simulink model "yuan_untitled_final_waveforms_SOM_PLL_fixed"  (R2023b)
settings: Solver=FixedStepDiscrete  StartTime=0.0  StopTime=0.5  FixedStep=1e-6  RelTol=1e-3
libraries: slpidlib x3, spsDCVoltageSourceLib x1, spsGroundLib x1, spsPermanentMagnetSynchronousMachineLib x1, spsThreePhaseVIMeasurementLib x1, spsUniversalBridgeLib x1, sps_lib x1
settings Model: Creator=zxw  LastModifiedBy=zxw

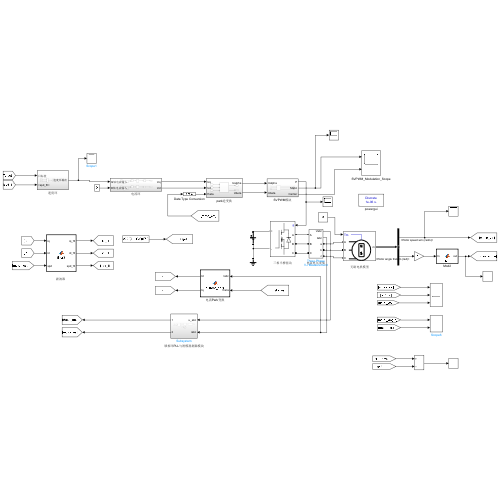
[thumbnail: Simulink's stored preview of the top-level diagram]
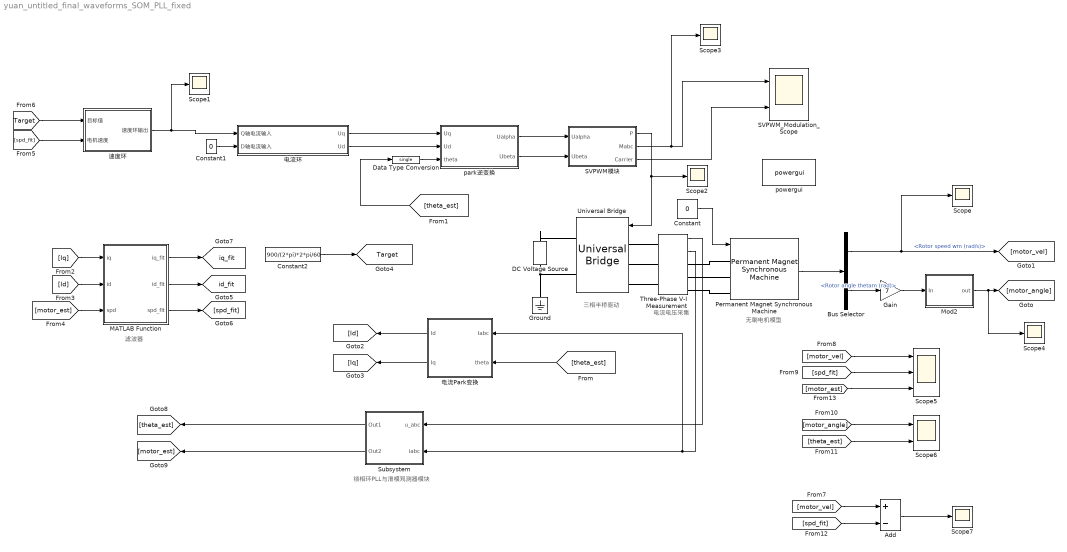
== system yuan_untitled_final_waveforms_SOM_PLL_fixed ==
  note: 锁相环PLL与滑模观测器模块
  note: 滤波器
  note: 无刷电机模型
  note: 电流电压采集
  note: 三相半桥驱动
  Add : Sum  Inputs=+-
  Bus Selector : BusSelector  OutputSignals=Rotor speed wm (rad/s),Rotor angle thetam (rad)
  Constant : Constant  Value=0
  Constant1 : Constant  Value=0
  Constant2 : Constant  Value=900/(2*pi)*2*pi/60
  DC Voltage Source : spsDCVoltageSourceLib/DC Voltage Source  Amplitude=24  Measurements=None
  Data Type Conversion : DataTypeConversion  OutDataTypeStr=single  RndMeth=Nearest  SaturateOnIntegerOverflow=off
  Gain : Gain  Gain=7
  Ground : spsGroundLib/Ground  LConnTagsString=a
  MATLAB Function : MATLAB Function  TreatAsAtomicUnit=on
  Mod2 : MATLAB Function  TreatAsAtomicUnit=on
  Permanent Magnet Synchronous Machine : spsPermanentMagnetSynchronousMachineLib/Permanent Magnet Synchronous Machine  NbPhases=3  FluxDistribution=Sinusoidal  RotorType=Round  MechanicalLoad=Torque Tm  PresetModel=No  ShowDetailedParameters=on  MeasurementBus=off  Resistance=0.0485  Inductance=8.5e-3  dqInductances=[8.5e-3,8.5e-3]  La=0.000395  MachineConstant=Flux linkage established by magnets (V.s)  Flux=0.1194  VoltageCst=151.5974  TorqueCst=1.2537  Flat=120  Mechanical=[0.0027 0.0004924 7 0]  PolePairs=4  InitialConditions=[0,0, 0,0]  InitialConditions5ph=[0 0 0 0 0 0]  RefAngle=90 degrees behind phase A axis (modified Park)  IterativeDiscreteModel=Trapezoidal non iterative  TsBlock=-1  TsPowergui=0
  SVPWM_Modulation_Scope : Scope  NumInputPorts=2
  SVPWM模块 : Subsystem
  Scope{,1..4,7} (6 alike) : Scope
  Scope5 : Scope  NumInputPorts=3
  Scope6 : Scope  NumInputPorts=2
  Subsystem : Subsystem
  Three-Phase V-I Measurement : spsThreePhaseVIMeasurementLib/Three-Phase V-I Measurement  VoltageMeasurement=phase-to-ground  SetLabelV=off  LabelV=Vabc  Vpu=off  VpuLL=off  CurrentMeasurement=yes  SetLabelI=off  LabelI=Iabc  Ipu=off  Pbase=100e6  Vbase=500e3  OutputType=Complex  PhasorSimulation=off  PSBequivalent=0
  Universal Bridge : spsUniversalBridgeLib/Universal Bridge  Arms=3  SnubberResistance=1e5  SnubberCapacitance=inf  Device=MOSFET / Diodes  Ron=1e-3  Lon=0  ForwardVoltages="[  0  0  ]"  ForwardVoltage=0  GTOparameters=[ 10e-6 , 20e-6 ]  IGBTparameters=[ 1e-6 , 2e-6 ]  Measurements=None  Measurements_2=None  converterType=Rectifier
  park逆变换 : Subsystem
  powergui : sps_lib/powergui  Priority=1  SimulationMode=Discrete  SampleTime=1e-6  frequency=60  Iterations=50  frequencyindice=0  Pbase=100e6  ErrMax=1e-4  UnitsV=kV  UnitsW=MW  buscounter=0  FunctionMessages=off  echomessages=off  EnableUseOfTLC=off  CurrentSourceSwitches=off  DisableSnubberDevices=off  DisableRonSwitches=off  DisableVfSwitches=off  DisplayEquations=off  AutomaticDiscreteSolvers=off  SolverType=Tustin/Backward Euler (TBE)  Interpol=off  ExternalGateDelay=off  methode=off  Ts=100  x0status=blocks  SPID=on  SwTol=0  HookPort=off  NonlinearTolerance=1e-4  nMaxIteration=100  ContinueOnMaxIteration=off  RestoreLinks=warning  ResistiveCurrentMeasurement=off  Frange=[0:2:500]  Ylog=off  Xlog=on  ShowGrid=off  save=off  variable=ZData  structure=0  ZoomFFT=off  StartTime=0.0  cycles=1  DisplayStyle=1  fundamental=60  FreqAxis=off  MaxFrequency=1000  frequencyindicesteady=1  RmsSteady=1  display=off
  电流Park变换 : MATLAB Function  TreatAsAtomicUnit=on
  电流环 : Subsystem
  速度环 : Subsystem
  tag scope: Target=global, id_fit=global, iq_fit=global
  wires:
  Permanent Magnet Synchronous Machine/1 -> Bus Selector/1
  Bus Selector/2 -> Gain/1  "<Rotor angle thetam (rad)>"
  Gain/1 -> Mod2/1(In)
  Mod2/1(out) -> Scope4/1, [motor_angle]
  Bus Selector/1 -> Scope/1, [motor_vel]  "<Rotor speed wm (rad/s)>"
  Constant/1 -> Permanent Magnet Synchronous Machine/1
  park逆变换/2(Ubeta) -> SVPWM模块/2(Ubeta)
  park逆变换/1(Ualpha) -> SVPWM模块/1(Ualpha)
  [theta_est] -> 电流Park变换/2(theta)
  Data Type Conversion/1 -> park逆变换/3(theta)
  [theta_est] -> Data Type Conversion/1
  电流Park变换/1(Id) -> [Id]
  电流Park变换/2(Iq) -> [Iq]
  [Iq] -> MATLAB Function/1(iq)
  [Id] -> MATLAB Function/2(id)
  [motor_est] -> MATLAB Function/3(spd)
  MATLAB Function/1(iq_flt) -> [iq_fit]
  MATLAB Function/2(id_flt) -> [id_fit]
  MATLAB Function/3(spd_flt) -> [spd_fit]
  电流环/2(Ud) -> park逆变换/2(Ud)
  电流环/1(Uq) -> park逆变换/1(Uq)
  Constant1/1 -> 电流环/2(D轴电流输入)
  Constant2/1 -> [Target]
  [Target] -> 速度环/1(目标值)
  [spd_fit] -> 速度环/2(电机速度)
  速度环/1(速度环输出) -> Scope1/1, 电流环/1(Q轴电流输入)
  SVPWM模块/2(Mabc) -> Scope3/1, SVPWM_Modulation_Scope/1
  SVPWM模块/3(Carrier) -> SVPWM_Modulation_Scope/2
  SVPWM模块/1(P) -> Scope2/1, Universal Bridge/1
  Three-Phase V-I Measurement/2 -> 电流Park变换/1(Iabc), Subsystem/2(iabc)
  [motor_vel] -> Scope5/1
  [spd_fit] -> Scope5/2
  [theta_est] -> Scope6/2
  [motor_angle] -> Scope6/1
  Three-Phase V-I Measurement/1 -> Subsystem/1(u_abc)
  Subsystem/1(Out1) -> [theta_est]
  Subsystem/2(Out2) -> [motor_est]
  [spd_fit] -> Add/2
  [motor_vel] -> Add/1
  Add/1 -> Scope7/1
  [motor_est] -> Scope5/3
  connections:
  Three-Phase V-I Measurement/RConn1 -- Permanent Magnet Synchronous Machine/LConn1
  Three-Phase V-I Measurement/RConn2 -- Permanent Magnet Synchronous Machine/LConn2
  Three-Phase V-I Measurement/RConn3 -- Permanent Magnet Synchronous Machine/LConn3
  Universal Bridge/LConn1 -- Three-Phase V-I Measurement/LConn1
  Universal Bridge/LConn2 -- Three-Phase V-I Measurement/LConn2
  Universal Bridge/LConn3 -- Three-Phase V-I Measurement/LConn3
  DC Voltage Source/RConn1 -- Universal Bridge/RConn1
  DC Voltage Source/LConn1 -- Universal Bridge/RConn2 -- Ground/LConn1

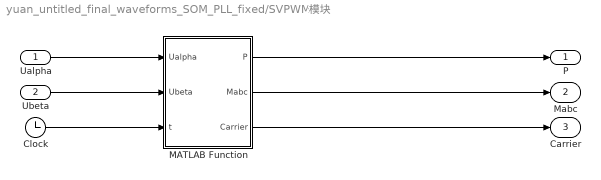
== system yuan_untitled_final_waveforms_SOM_PLL_fixed/SVPWM模块 ==
  Ualpha : Inport
  Ubeta : Inport  Port=2
  Clock : Clock
  MATLAB Function : MATLAB Function  TreatAsAtomicUnit=on
  P : Outport
  Mabc : Outport  Port=2
  Carrier : Outport  Port=3
  wires:
  Ualpha/1 -> MATLAB Function/1(Ualpha)
  MATLAB Function/1(P) -> P/1
  Ubeta/1 -> MATLAB Function/2(Ubeta)
  Clock/1 -> MATLAB Function/3(t)
  MATLAB Function/2(Mabc) -> Mabc/1
  MATLAB Function/3(Carrier) -> Carrier/1

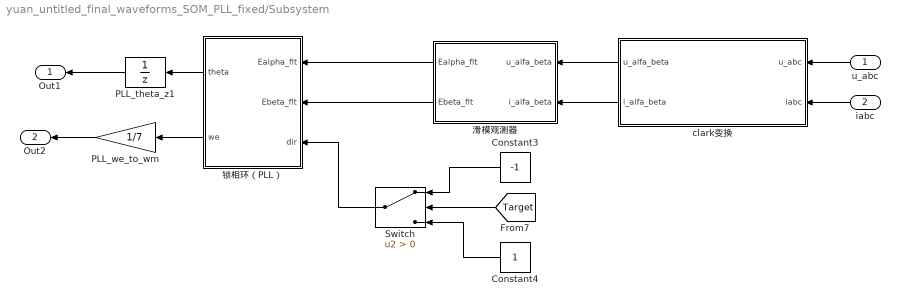
== system yuan_untitled_final_waveforms_SOM_PLL_fixed/Subsystem ==
  u_abc : Inport
  iabc : Inport  Port=2
  Constant3 : Constant  Value=-1
  Constant4 : Constant
  PLL_theta_z1 : UnitDelay  SampleTime=1e-6  HasFrameUpgradeWarning=on
  PLL_we_to_wm : Gain  Gain=1/7
  Switch : Switch  Criteria=u2 > Threshold  SaturateOnIntegerOverflow=off  InputSameDT=off
  clark变换 : MATLAB Function  TreatAsAtomicUnit=on
  滑模观测器 : MATLAB Function  TreatAsAtomicUnit=on
  锁相环（PLL） : MATLAB Function  TreatAsAtomicUnit=on
  Out1 : Outport
  Out2 : Outport  Port=2
  wires:
  PLL_we_to_wm/1 -> Out2/1
  clark变换/2(i_alfa_beta) -> 滑模观测器/2(i_alfa_beta)
  clark变换/1(u_alfa_beta) -> 滑模观测器/1(u_alfa_beta)
  滑模观测器/2(Ebeta_flt) -> 锁相环（PLL）/2(Ebeta_flt)
  Constant3/1 -> Switch/1
  滑模观测器/1(Ealpha_flt) -> 锁相环（PLL）/1(Ealpha_flt)
  Constant4/1 -> Switch/3
  Switch/1 -> 锁相环（PLL）/3(dir)
  [Target] -> Switch/2
  锁相环（PLL）/1(theta) -> PLL_theta_z1/1
  锁相环（PLL）/2(we) -> PLL_we_to_wm/1
  PLL_theta_z1/1 -> Out1/1
  iabc/1 -> clark变换/2(iabc)
  u_abc/1 -> clark变换/1(u_abc)

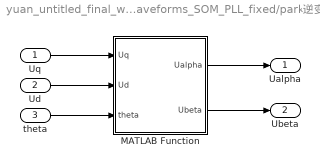
== system yuan_untitled_final_waveforms_SOM_PLL_fixed/park逆变换 ==
  Uq : Inport
  Ud : Inport  Port=2
  theta : Inport  Port=3
  MATLAB Function : MATLAB Function  TreatAsAtomicUnit=on
  Ualpha : Outport
  Ubeta : Outport  Port=2
  wires:
  MATLAB Function/1(Ualpha) -> Ualpha/1
  MATLAB Function/2(Ubeta) -> Ubeta/1
  Uq/1 -> MATLAB Function/1(Uq)
  Ud/1 -> MATLAB Function/2(Ud)
  theta/1 -> MATLAB Function/3(theta)

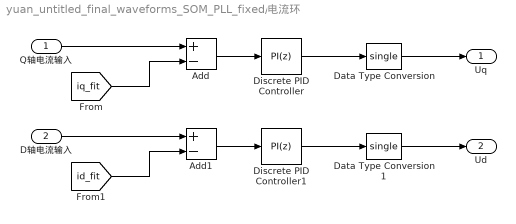
== system yuan_untitled_final_waveforms_SOM_PLL_fixed/电流环 ==
  Q轴电流输入 : Inport
  D轴电流输入 : Inport  Port=2
  Add : Sum  Inputs=+-
  Add1 : Sum  Inputs=+-
  Data Type Conversion : DataTypeConversion  OutDataTypeStr=single  RndMeth=Nearest  SaturateOnIntegerOverflow=off
  Data Type Conversion1 : DataTypeConversion  OutDataTypeStr=single  RndMeth=Nearest  SaturateOnIntegerOverflow=off
  Discrete PID Controller : slpidlib/PID Controller  Controller=PI  Form=Parallel  TimeDomain=Discrete-time  UseExternalTs=off  SampleTime=1e-4  IntegratorMethod=Forward Euler  FilterMethod=Forward Euler  ControllerParametersSource=internal  P=5.34  I=30.47  UseKiTs=off  D=0  N=100  UseFilter=on  TunerSelectOption=Transfer Function Based (PID Tuner App)  InitialConditionSource=internal  InitialConditionForIntegrator=0  InitialConditionForFilter=0  DifferentiatorICPrevScaledInput=0  ExternalReset=none  TrackingMode=off  Kt=1  LimitOutput=on  SatLimitsSource=internal  UpperSaturationLimit=24/sqrt(3)  LowerSaturationLimit=-24/sqrt(3)  LinearizeAsGain=off  AntiWindupMode=back-calculation  Kb=100  LimitIntegrator=off  UpperIntegratorSaturationLimit=inf  LowerIntegratorSaturationLimit=-inf  POutMin=[]  POutMax=[]  IOutMin=[]  IOutMax=[]  DOutMin=[]  DOutMax=[]  NOutMin=[]  NOutMax=[]  SumOutMin=[]  SumOutMax=[]  SaturationOutMin=[]  SaturationOutMax=[]  PParamMin=[]  PParamMax=[]  IParamMin=[]  IParamMax=[]  DParamMin=[]  DParamMax=[]  NParamMin=[]  NParamMax=[]  KbParamMin=[]  KbParamMax=[]  KtParamMin=[]  KtParamMax=[]  KbOutMin=[]  KbOutMax=[]  KtOutMin=[]  KtOutMax=[]  IntegratorOutMin=[]  IntegratorOutMax=[]  FilterOutMin=[]  FilterOutMax=[]  SumI1OutMin=[]  SumI1OutMax=[]  SumI2OutMin=[]  SumI2OutMax=[]  SumI3OutMin=[]  SumI3OutMax=[]  SumI4OutMin=[]  SumI4OutMax=[]  SumDOutMin=[]  SumDOutMax=[]  DifferentiatorOutMin=[]  DifferentiatorOutMax=[]  FilterDiffOutCoefMin=[]  FilterDiffOutCoefMax=[]  ReciprocalOutMin=[]  ReciprocalOutMax=[]  SumDenOutMin=[]  SumDenOutMax=[]  SumNumOutMin=[]  SumNumOutMax=[]  DivideOutMin=[]  DivideOutMax=[]  UdiffTsProdOutMin=[]  UdiffTsProdOutMax=[]  NTsProdOutMin=[]  NTsProdOutMax=[]  UintegralTsProdOutMin=[]  UintegralTsProdOutMax=[]  UngainTsProdOutMin=[]  UngainTsProdOutMax=[]  ClampingZeroOutDataTypeStr=Inherit: Inherit via back propagation  ClampingZeroOutMin=[]  ClampingZeroOutMax=[]  FilterDenConstantOutDataTypeStr=Inherit: Inherit via back propagation  FilterDenConstantOutMin=[]  FilterDenConstantOutMax=[]  PCopyOutDataTypeStr=Inherit: Inherit via back propagation  PCopyOutMin=[]  PCopyOutMax=[]  NCopyOutDataTypeStr=Inherit: Inherit via back propagation  NCopyOutMin=[]  NCopyOutMax=[]  IntegratorContinuousStateAttributes=''  IntegratorStateMustResolveToSignalObject=off  IntegratorRTWStateStorageClass=Auto  FilterContinuousStateAttributes=''  FilterStateMustResolveToSignalObject=off  FilterRTWStateStorageClass=Auto  ParallelPVariant=InternalParameters  IdealPVariant=Disabled  IVariant=InternalParameters  DVariant=Disabled  IntegratorVariant=Discrete  SatVariant=Enabled  AWVariant=BackCalculation  PCopyVariant=Disabled  TRVariant=Disabled  FdbkBlocksVariant=Forward  IdealPFdbkVariant=Disabled  SatFdbkVariant=Disabled  DerivativeFilterVariant=Disabled  NVariant=Disabled  NCopyVariant=Disabled_SignalSpec  FilterICVariant=Disabled  IntegratorICVariant=InternalICs  ExternalResetVariant=Disabled  TRSumVariant=Passthrough  SumFdbkVariant=Disabled  SumVariant=Sum_PI  TsampFilterVariant=InternalTs  TsampNgainVariant=Passthrough  TsampIntegralVariant=Disabled_SignalSpec  ExternalSaturationOutDataTypeStr=Inherit: Same as second input
      settings: LibrarySourceBlock=|
      | hdlsllib/HDL Floating Point
      | Operations/Discrete PID Controller
  Discrete PID Controller1 : slpidlib/PID Controller  Controller=PI  Form=Parallel  TimeDomain=Discrete-time  UseExternalTs=off  SampleTime=1e-4  IntegratorMethod=Forward Euler  FilterMethod=Forward Euler  ControllerParametersSource=internal  P=5.34  I=30.47  UseKiTs=off  D=0  N=100  UseFilter=on  TunerSelectOption=Transfer Function Based (PID Tuner App)  InitialConditionSource=internal  InitialConditionForIntegrator=0  InitialConditionForFilter=0  DifferentiatorICPrevScaledInput=0  ExternalReset=none  TrackingMode=off  Kt=1  LimitOutput=on  SatLimitsSource=internal  UpperSaturationLimit=24/sqrt(3)  LowerSaturationLimit=-24/sqrt(3)  LinearizeAsGain=off  AntiWindupMode=back-calculation  Kb=100  LimitIntegrator=off  UpperIntegratorSaturationLimit=inf  LowerIntegratorSaturationLimit=-inf  POutMin=[]  POutMax=[]  IOutMin=[]  IOutMax=[]  DOutMin=[]  DOutMax=[]  NOutMin=[]  NOutMax=[]  SumOutMin=[]  SumOutMax=[]  SaturationOutMin=[]  SaturationOutMax=[]  PParamMin=[]  PParamMax=[]  IParamMin=[]  IParamMax=[]  DParamMin=[]  DParamMax=[]  NParamMin=[]  NParamMax=[]  KbParamMin=[]  KbParamMax=[]  KtParamMin=[]  KtParamMax=[]  KbOutMin=[]  KbOutMax=[]  KtOutMin=[]  KtOutMax=[]  IntegratorOutMin=[]  IntegratorOutMax=[]  FilterOutMin=[]  FilterOutMax=[]  SumI1OutMin=[]  SumI1OutMax=[]  SumI2OutMin=[]  SumI2OutMax=[]  SumI3OutMin=[]  SumI3OutMax=[]  SumI4OutMin=[]  SumI4OutMax=[]  SumDOutMin=[]  SumDOutMax=[]  DifferentiatorOutMin=[]  DifferentiatorOutMax=[]  FilterDiffOutCoefMin=[]  FilterDiffOutCoefMax=[]  ReciprocalOutMin=[]  ReciprocalOutMax=[]  SumDenOutMin=[]  SumDenOutMax=[]  SumNumOutMin=[]  SumNumOutMax=[]  DivideOutMin=[]  DivideOutMax=[]  UdiffTsProdOutMin=[]  UdiffTsProdOutMax=[]  NTsProdOutMin=[]  NTsProdOutMax=[]  UintegralTsProdOutMin=[]  UintegralTsProdOutMax=[]  UngainTsProdOutMin=[]  UngainTsProdOutMax=[]  ClampingZeroOutDataTypeStr=Inherit: Inherit via back propagation  ClampingZeroOutMin=[]  ClampingZeroOutMax=[]  FilterDenConstantOutDataTypeStr=Inherit: Inherit via back propagation  FilterDenConstantOutMin=[]  FilterDenConstantOutMax=[]  PCopyOutDataTypeStr=Inherit: Inherit via back propagation  PCopyOutMin=[]  PCopyOutMax=[]  NCopyOutDataTypeStr=Inherit: Inherit via back propagation  NCopyOutMin=[]  NCopyOutMax=[]  IntegratorContinuousStateAttributes=''  IntegratorStateMustResolveToSignalObject=off  IntegratorRTWStateStorageClass=Auto  FilterContinuousStateAttributes=''  FilterStateMustResolveToSignalObject=off  FilterRTWStateStorageClass=Auto  ParallelPVariant=InternalParameters  IdealPVariant=Disabled  IVariant=InternalParameters  DVariant=Disabled  IntegratorVariant=Discrete  SatVariant=Enabled  AWVariant=BackCalculation  PCopyVariant=Disabled  TRVariant=Disabled  FdbkBlocksVariant=Forward  IdealPFdbkVariant=Disabled  SatFdbkVariant=Disabled  DerivativeFilterVariant=Disabled  NVariant=Disabled  NCopyVariant=Disabled_SignalSpec  FilterICVariant=Disabled  IntegratorICVariant=InternalICs  ExternalResetVariant=Disabled  TRSumVariant=Passthrough  SumFdbkVariant=Disabled  SumVariant=Sum_PI  TsampFilterVariant=InternalTs  TsampNgainVariant=Passthrough  TsampIntegralVariant=Disabled_SignalSpec  ExternalSaturationOutDataTypeStr=Inherit: Same as second input
      settings: LibrarySourceBlock=|
      | hdlsllib/HDL Floating Point
      | Operations/Discrete PID Controller
  Uq : Outport
  Ud : Outport  Port=2
  wires:
  Q轴电流输入/1 -> Add/1
  [iq_fit] -> Add/2
  D轴电流输入/1 -> Add1/1
  [id_fit] -> Add1/2
  Add/1 -> Discrete PID Controller/1
  Add1/1 -> Discrete PID Controller1/1
  Discrete PID Controller/1 -> Data Type Conversion/1
  Data Type Conversion/1 -> Uq/1
  Discrete PID Controller1/1 -> Data Type Conversion1/1
  Data Type Conversion1/1 -> Ud/1

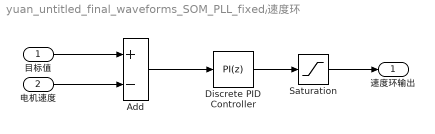
== system yuan_untitled_final_waveforms_SOM_PLL_fixed/速度环 ==
  目标值 : Inport
  电机速度 : Inport  Port=2
  Add : Sum  Inputs=+-
  Discrete PID Controller : slpidlib/PID Controller  Controller=PI  Form=Parallel  TimeDomain=Discrete-time  UseExternalTs=off  SampleTime=1e-3  IntegratorMethod=Forward Euler  FilterMethod=Forward Euler  ControllerParametersSource=internal  P=0.334  I=14.88  UseKiTs=off  D=0  N=100  UseFilter=on  TunerSelectOption=Transfer Function Based (PID Tuner App)  InitialConditionSource=internal  InitialConditionForIntegrator=0  InitialConditionForFilter=0  DifferentiatorICPrevScaledInput=0  ExternalReset=none  TrackingMode=off  Kt=1  LimitOutput=on  SatLimitsSource=internal  UpperSaturationLimit=5  LowerSaturationLimit=-5  LinearizeAsGain=off  AntiWindupMode=back-calculation  Kb=50  LimitIntegrator=off  UpperIntegratorSaturationLimit=inf  LowerIntegratorSaturationLimit=-inf  POutMin=[]  POutMax=[]  IOutMin=[]  IOutMax=[]  DOutMin=[]  DOutMax=[]  NOutMin=[]  NOutMax=[]  SumOutMin=[]  SumOutMax=[]  SaturationOutMin=[]  SaturationOutMax=[]  PParamMin=[]  PParamMax=[]  IParamMin=[]  IParamMax=[]  DParamMin=[]  DParamMax=[]  NParamMin=[]  NParamMax=[]  KbParamMin=[]  KbParamMax=[]  KtParamMin=[]  KtParamMax=[]  KbOutMin=[]  KbOutMax=[]  KtOutMin=[]  KtOutMax=[]  IntegratorOutMin=[]  IntegratorOutMax=[]  FilterOutMin=[]  FilterOutMax=[]  SumI1OutMin=[]  SumI1OutMax=[]  SumI2OutMin=[]  SumI2OutMax=[]  SumI3OutMin=[]  SumI3OutMax=[]  SumI4OutMin=[]  SumI4OutMax=[]  SumDOutMin=[]  SumDOutMax=[]  DifferentiatorOutMin=[]  DifferentiatorOutMax=[]  FilterDiffOutCoefMin=[]  FilterDiffOutCoefMax=[]  ReciprocalOutMin=[]  ReciprocalOutMax=[]  SumDenOutMin=[]  SumDenOutMax=[]  SumNumOutMin=[]  SumNumOutMax=[]  DivideOutMin=[]  DivideOutMax=[]  UdiffTsProdOutMin=[]  UdiffTsProdOutMax=[]  NTsProdOutMin=[]  NTsProdOutMax=[]  UintegralTsProdOutMin=[]  UintegralTsProdOutMax=[]  UngainTsProdOutMin=[]  UngainTsProdOutMax=[]  ClampingZeroOutDataTypeStr=Inherit: Inherit via back propagation  ClampingZeroOutMin=[]  ClampingZeroOutMax=[]  FilterDenConstantOutDataTypeStr=Inherit: Inherit via back propagation  FilterDenConstantOutMin=[]  FilterDenConstantOutMax=[]  PCopyOutDataTypeStr=Inherit: Inherit via back propagation  PCopyOutMin=[]  PCopyOutMax=[]  NCopyOutDataTypeStr=Inherit: Inherit via back propagation  NCopyOutMin=[]  NCopyOutMax=[]  IntegratorContinuousStateAttributes=''  IntegratorStateMustResolveToSignalObject=off  IntegratorRTWStateStorageClass=Auto  FilterContinuousStateAttributes=''  FilterStateMustResolveToSignalObject=off  FilterRTWStateStorageClass=Auto  ParallelPVariant=InternalParameters  IdealPVariant=Disabled  IVariant=InternalParameters  DVariant=Disabled  IntegratorVariant=Discrete  SatVariant=Enabled  AWVariant=BackCalculation  PCopyVariant=Disabled  TRVariant=Disabled  FdbkBlocksVariant=Forward  IdealPFdbkVariant=Disabled  SatFdbkVariant=Disabled  DerivativeFilterVariant=Disabled  NVariant=Disabled  NCopyVariant=Disabled_SignalSpec  FilterICVariant=Disabled  IntegratorICVariant=InternalICs  ExternalResetVariant=Disabled  TRSumVariant=Passthrough  SumFdbkVariant=Disabled  SumVariant=Sum_PI  TsampFilterVariant=InternalTs  TsampNgainVariant=Passthrough  TsampIntegralVariant=Disabled_SignalSpec  ExternalSaturationOutDataTypeStr=Inherit: Same as second input
      settings: LibrarySourceBlock=simulink/Discrete/Discrete PID Controller
  Saturation : Saturate  UpperLimit=10  LowerLimit=-10
  速度环输出 : Outport
  wires:
  电机速度/1 -> Add/2
  目标值/1 -> Add/1
  Add/1 -> Discrete PID Controller/1
  Discrete PID Controller/1 -> Saturation/1
  Saturation/1 -> 速度环输出/1

== matlab function yuan_untitled_final_waveforms_SOM_PLL_fixed/SVPWM模块/MATLAB Function ==
  data: Ualpha input; P output; Ubeta input; t input; Mabc output; Carrier output
function [P, Mabc, Carrier] = svpwm(Ualpha, Ubeta, t)
% 输入：Ualpha、Ubeta，单位V
% 输出：[A上 A下 B上 B下 C上 C下]

Vdc = 24;       % 直流母线电压
Fsw = 10000;    % 开关频率10 kHz

% 逆Clarke变换：alpha-beta转三相参考电压
Va = Ualpha;
Vb = -0.5*Ualpha + sqrt(3)/2*Ubeta;
Vc = -0.5*Ualpha - sqrt(3)/2*Ubeta;

% 判断是否超出SVPWM线性范围
% 两电平逆变器能够产生的最大线电压范围为Vdc，因此必须满足：Vmax - Vmin < Vdc
Vmax = max(Va, max(Vb, Vc));
Vmin = min(Va, min(Vb, Vc));
Vspan = Vmax - Vmin;

if Vspan > Vdc
    K = Vdc/Vspan;
    Va = K*Va;
    Vb = K*Vb;
    Vc = K*Vc;

    Vmax = max(Va, max(Vb, Vc));
    Vmin = min(Va, min(Vb, Vc));
end

% 零序电压注入
Vzero = -0.5*(Vmax + Vmin);

% 三相占空比
Da = 0.5 + (Va + Vzero)/Vdc;
Db = 0.5 + (Vb + Vzero)/Vdc;
Dc = 0.5 + (Vc + Vzero)/Vdc;

Da = min(max(Da,0),1);
Db = min(max(Db,0),1);
Dc = min(max(Dc,0),1);

% % 生成0~1中心对齐三角载波
% carrierPhase = mod(t*Fsw,1);
% carrier = 1 - abs(2*carrierPhase - 1);

% 两端为1、中心为0的对称三角载波
carrierPhase = mod(t*Fsw, 1);
carrier = abs(2*carrierPhase - 1);

% Normalized SVPWM modulation waves and bipolar carrier for display
Mabc = zeros(3,1);
Mabc(1) = 2*Da - 1;
Mabc(2) = 2*Db - 1;
Mabc(3) = 2*Dc - 1;
Carrier = 2*carrier - 1;

Sa = double(Da > carrier);
Sb = double(Db > carrier);
Sc = double(Dc > carrier);

% 处理0%和100%占空比
if Da <= 0
    Sa = 0;
elseif Da >= 1
    Sa = 1;
end

if Db <= 0
    Sb = 0;
elseif Db >= 1
    Sb = 1;
end

if Dc <= 0
    Sc = 0;
elseif Dc >= 1
    Sc = 1;
end

% 六路桥臂驱动信号
P = zeros(6,1);
P(1) = Sa;       % A相上管
P(2) = 1-Sa;     % A相下管
P(3) = Sb;       % B相上管
P(4) = 1-Sb;     % B相下管
P(5) = Sc;       % C相上管
P(6) = 1-Sc;     % C相下管
end

== matlab function yuan_untitled_final_waveforms_SOM_PLL_fixed/Mod2 ==
  data: In input; out output
function out = fcn(In)
out = mod(In, 2*pi);
end

== matlab function yuan_untitled_final_waveforms_SOM_PLL_fixed/park逆变换/MATLAB Function ==
  data: Uq input; Ualpha output; Ud input; theta input; Ubeta output
function [Ualpha, Ubeta] = inverse_park(Uq, Ud, theta)
% Inverse Park matching phase-a to q-axis convention
c = cos(theta);
s = sin(theta);
Ualpha = Uq*c + Ud*s;
Ubeta  = Uq*s - Ud*c;
end

== matlab function yuan_untitled_final_waveforms_SOM_PLL_fixed/电流Park变换 ==
  data: Iabc input; Id output; theta input; Iq output
function [Id, Iq] = current_park(Iabc, theta)
% Clarke + Park, phase-a aligned with q-axis
Ia = Iabc(1);
Ib = Iabc(2);
Ic = Iabc(3);
Ialpha = (2/3)*(Ia - 0.5*Ib - 0.5*Ic);
Ibeta  = (2/3)*(sqrt(3)/2)*(Ib - Ic);
c = cos(theta);
s = sin(theta);
Iq = Ialpha*c + Ibeta*s;
Id = Ialpha*s - Ibeta*c;
end

== matlab function yuan_untitled_final_waveforms_SOM_PLL_fixed/MATLAB Function ==
  settings: updateMethod=DISCRETE
  data: iq input; iq_flt output; id input; spd input; id_flt output; spd_flt output
function [iq_flt, id_flt, spd_flt] = filter3(iq, id, spd)
% iq、id和转速的一阶低通滤波器

% 实际执行周期
Ts = 1e-4;

% 截止频率
Fc_current = 2000;  % dq电流截止频率：2 kHz
Fc_speed   = 100;   % 转速截止频率：100 Hz

% 离散滤波系数
Alpha_current = 1 - exp(-2*pi*Fc_current*Ts);
Alpha_speed   = 1 - exp(-2*pi*Fc_speed*Ts);

% 滤波器内部状态
persistent iq_state id_state spd_state initialized

if isempty(initialized)
    % 使用第一次采样值初始化，避免启动跳变
    iq_state  = iq;
    id_state  = id;
    spd_state = spd;
    initialized = true;
end

% dq电流低通滤波
iq_state = iq_state + Alpha_current*(iq - iq_state);
id_state = id_state + Alpha_current*(id - id_state);

% 速度低通滤波
spd_state = spd_state + Alpha_speed*(spd - spd_state);

% 输出
iq_flt  = iq_state;
id_flt  = id_state;
spd_flt = spd_state;
end

== matlab function yuan_untitled_final_waveforms_SOM_PLL_fixed/Subsystem/clark变换 ==
  data: u_abc input; u_alfa_beta output; iabc input; i_alfa_beta output
function [u_alfa_beta, i_alfa_beta] = clarke_transform(u_abc, iabc)
%#codegen
% 输入：
%   u_abc = [Ua; Ub; Uc]
%   iabc  = [Ia; Ib; Ic]
%
% 输出：
%   u_alfa_beta = [Ualpha; Ubeta]
%   i_alfa_beta = [Ialpha; Ibeta]

Ua = u_abc(1);
Ub = u_abc(2);
Uc = u_abc(3);

Ia = iabc(1);
Ib = iabc(2);
Ic = iabc(3);

% 电压 Clarke 变换
Ualpha = (2/3) * (Ua - 0.5*Ub - 0.5*Uc);
Ubeta  = (2/3) * (sqrt(3)/2) * (Ub - Uc);

% 电流 Clarke 变换
Ialpha = (2/3) * (Ia - 0.5*Ib - 0.5*Ic);
Ibeta  = (2/3) * (sqrt(3)/2) * (Ib - Ic);

% 二维列向量输出
u_alfa_beta = [Ualpha; Ubeta];
i_alfa_beta = [Ialpha; Ibeta];

end

== matlab function yuan_untitled_final_waveforms_SOM_PLL_fixed/Subsystem/滑模观测器 ==
  data: u_alfa_beta input; Ealpha_flt output; i_alfa_beta input; Ebeta_flt output
function [Ealpha_flt, Ebeta_flt] = SMO(u_alfa_beta, i_alfa_beta)
%#codegen
Ts = 1e-6;
Rs = 0.0485;
Ls = 8.5e-3;
Ksw = 18;
boundary = 0.5;
Fc_emf = 500;
emf_a = exp(-2*pi*Fc_emf*Ts);

Ualpha = u_alfa_beta(1);
Ubeta  = u_alfa_beta(2);
Ialpha = i_alfa_beta(1);
Ibeta  = i_alfa_beta(2);

persistent Ihat_alpha_state Ihat_beta_state
persistent Ealpha_state Ebeta_state
persistent Ealpha_flt_state Ebeta_flt_state

if isempty(Ihat_alpha_state)
    Ihat_alpha_state = 0;
    Ihat_beta_state = 0;
    Ealpha_state = 0;
    Ebeta_state = 0;
    Ealpha_flt_state = 0;
    Ebeta_flt_state = 0;
end

dIhat_alpha = (Ualpha - Rs*Ihat_alpha_state - Ealpha_state)/Ls;
dIhat_beta  = (Ubeta  - Rs*Ihat_beta_state  - Ebeta_state )/Ls;
Ihat_alpha_state = Ihat_alpha_state + Ts*dIhat_alpha;
Ihat_beta_state  = Ihat_beta_state  + Ts*dIhat_beta;

Ialpha_error = Ihat_alpha_state - Ialpha;
Ibeta_error  = Ihat_beta_state  - Ibeta;
sat_alpha = min(max(Ialpha_error/boundary, -1), 1);
sat_beta  = min(max(Ibeta_error /boundary, -1), 1);
Ealpha_state = Ksw*sat_alpha;
Ebeta_state  = Ksw*sat_beta;

Ealpha_flt_state = emf_a*Ealpha_flt_state + (1-emf_a)*Ealpha_state;
Ebeta_flt_state  = emf_a*Ebeta_flt_state  + (1-emf_a)*Ebeta_state;
Ealpha_flt = Ealpha_flt_state;
Ebeta_flt  = Ebeta_flt_state;
end

== matlab function yuan_untitled_final_waveforms_SOM_PLL_fixed/Subsystem/锁相环（PLL） ==
  data: Ealpha_flt input; theta output; Ebeta_flt input; dir input; we output
function [theta, we] = PLL(Ealpha_flt, Ebeta_flt, dir)
%#codegen
Ts = 1e-6;
PLL_kp = 35;
PLL_ki = 1400;
we_limit = 2000;
Emin = 0.5;
Fc_speed = 200;
speed_a = exp(-2*pi*Fc_speed*Ts);
Fc_emf = 500;
wc_emf = 2*pi*Fc_emf;

persistent theta_state integral_state we_flt
if isempty(theta_state)
    theta_state = pi/2;
    integral_state = 0;
    we_flt = 0;
end

if dir >= 0
    direction = 1;
else
    direction = -1;
end

Eamp = sqrt(Ealpha_flt^2 + Ebeta_flt^2);
if Eamp > Emin
    theta_error = direction*(-Ealpha_flt*cos(theta_state) ...
                                  -Ebeta_flt*sin(theta_state));
    integral_state = integral_state + Ts*PLL_ki*theta_error;
    integral_state = min(max(integral_state, -we_limit), we_limit);
    we_raw = PLL_kp*theta_error + integral_state;
    we_raw = min(max(we_raw, -we_limit), we_limit);
    theta_state = mod(theta_state + Ts*we_raw, 2*pi);
    we_flt = speed_a*we_flt + (1-speed_a)*we_raw;
end

phase_comp = atan(we_flt/wc_emf);
theta = mod(theta_state - pi/2 + phase_comp, 2*pi);
we = we_flt;
end
